simulink model "adc"  (R2019a)
settings: Solver=VariableStepAuto  StartTime=0.0  StopTime=500  RelTol=1e-3
libraries: xbsIndex_r4 x104, simulink x16
settings Model: Creator=qwerty40  LastModifiedBy=jackh
settings DataIOCC: ReturnWorkspaceOutputs=off
settings DebuggingCC: ArithmeticOperatorsInVariantConditions=warning
settings SFSimCC: SimUseLocalCustomCode=off
settings RTWCC: RTWUseLocalCustomCode=off
settings CodeAppCC: StateflowObjectComments=on

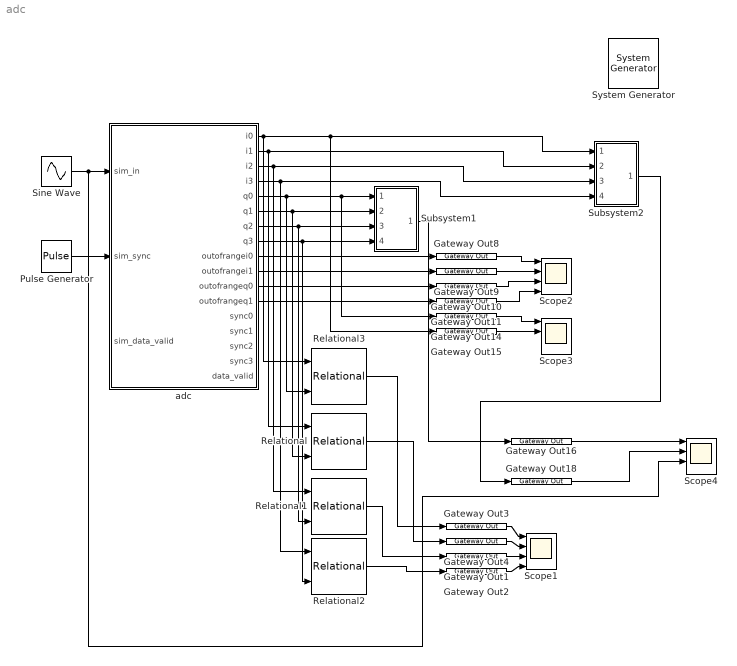
== system adc ==
  " System Generator" : xbsIndex_r4/ System Generator  Tag=genX  xilinxfamily=kintex7  part=xc7k325t  speed=-3  package=fbg676  synthesis_tool=Vivado  clock_wrapper=Clock Enables  directory=./netlist  proj_type=Vivado  Synth_file=Vivado Synthesis Defaults  Impl_file=Vivado Implementation Defaults  testbench=off  simulink_period=1  sysclk_period=10  dcm_input_clock_period=10  incr_netlist=off  trim_vbits=Everywhere in SubSystem  dbl_ovrd=According to Block Masks  core_generation=According to Block Masks  run_coregen=off  deprecated_control=off  eval_field=0  block_type=sysgen
  Gateway Out{1..4,8..11,14..16,18} (12 alike) : xbsIndex_r4/Gateway Out  inherit_from_input=off  hdl_port=on  rows=1  columns=1  UseAsDAC=off  DACChannel='1'  interface=None  automatic_assignment=on  address_offset=hex2dec('00')  intf_name=''  intf_description=''  timing_constraint=None  locs_specified=off  LOCs={}  io_standard={}  block_type=gatewayout
  Pulse Generator : DiscretePulseGenerator  Period=100
  Relational{,1..3} (4 alike) : xbsIndex_r4/Relational  mode=a=b  op_type=Bool  en=off  latency=1  dbl_ovrd=off  block_type=relational
  Scope{1..4} (4 alike) : Scope  NumInputPorts=4
  Sine Wave : Sin  SineType=Sample based  Amplitude=0.5  Frequency=pi / 30  Samples=100  SampleTime=1
  Subsystem1 : Subsystem
  Subsystem2 : Subsystem
  adc : Subsystem  Tag=xps:adc  mask(adc){adc_brd=adc0, adc_clk_rate=800, adc_interleave=off, sample_period=4}
      mask prompts: adc_brd "ADC board"; adc_clk_rate "ADC clock rate (MHz)"; adc_interleave "ADC interleave mode"; sample_period "Sample period"
      mask help: The ADC block converts analog inputs to digital outputs. Every clock cycle, the inputs are sampled and digitized to 8 bit binary point numbers in the range of [-1, 1) and are then output by the adc.
      mask init:
      | adc_mask;
      mask Help: eval('xlWeb([getenv(''MLIB_ROOT''), ''\doc\html\sys_adc\sys_adc.html''])')
      mask TypeOptions adc_brd: adc0 | adc1
  wires:
  Pulse Generator/1 -> adc/2(sim_sync)
  Gateway Out8/1 -> Scope2/1
  Gateway Out9/1 -> Scope2/2
  Gateway Out10/1 -> Scope2/3
  Gateway Out11/1 -> Scope2/4
  ? -> Scope3/4
  ? -> Scope3/3
  Gateway Out15/1 -> Scope3/2
  Gateway Out14/1 -> Scope3/1
  Gateway Out16/1 -> Scope4/1
  adc/1(i0) -> Relational3/1, Gateway Out15/1, Subsystem2/1(In1)
  adc/2(i1) -> Relational/1, Subsystem2/2(In2)
  adc/3(i2) -> Relational1/1, Subsystem2/3(In3)
  adc/4(i3) -> Relational2/1, Subsystem2/4(In4)
  Gateway Out18/1 -> Scope4/2
  adc/9(outofrangei0) -> Gateway Out8/1
  adc/10(outofrangei1) -> Gateway Out9/1
  adc/11(outofrangeq0) -> Gateway Out10/1
  adc/12(outofrangeq1) -> Gateway Out11/1
  Subsystem1/1(Out1) -> Gateway Out16/1
  Subsystem2/1(Out1) -> Gateway Out18/1
  adc/6(q1) -> Relational/2, Subsystem1/2(In2)
  adc/7(q2) -> Relational1/2, Subsystem1/3(In3)
  adc/8(q3) -> Relational2/2, Subsystem1/4(In4)
  adc/5(q0) -> Relational3/2, Subsystem1/1(In1), Gateway Out14/1
  Relational3/1 -> Gateway Out3/1
  Gateway Out3/1 -> Scope1/1
  Gateway Out4/1 -> Scope1/2
  Gateway Out1/1 -> Scope1/3
  Gateway Out2/1 -> Scope1/4
  Relational/1 -> Gateway Out4/1
  Relational1/1 -> Gateway Out1/1
  Relational2/1 -> Gateway Out2/1
  Sine Wave/1 -> Scope4/3, adc/1(sim_in)

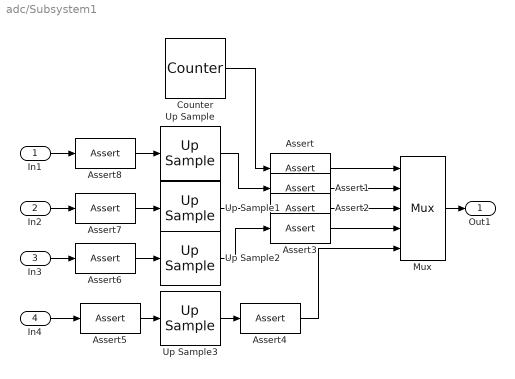
== system adc/Subsystem1 ==
  In1 : Inport
  In2 : Inport  Port=2
  In3 : Inport  Port=3
  In4 : Inport  Port=4
  Assert{,1..4} (5 alike) : xbsIndex_r4/Assert  assert_type=off  type_source=Explicitly  gui_display_data_type=Fixed-point  arith_type="Signed  (2's comp)"  n_bits=16  bin_pt=14  preci_type=Single  exp_width=8  frac_width=24  assert_rate=on  rate_source=Explicitly  period=1  output_port=on  block_type=assert
  Assert{5..8} (4 alike) : xbsIndex_r4/Assert  assert_type=off  type_source=Explicitly  gui_display_data_type=Fixed-point  arith_type="Signed  (2's comp)"  n_bits=16  bin_pt=14  preci_type=Single  exp_width=8  frac_width=24  assert_rate=on  rate_source=Explicitly  period=4  output_port=on  block_type=assert
  Counter : xbsIndex_r4/Counter  cnt_type=Free Running  cnt_to=Inf  operation=Up  start_count=0  cnt_by_val=1  arith_type=Unsigned  n_bits=2  bin_pt=0  load_pin=off  rst=off  en=off  explicit_period=on  period=1  use_behavioral_HDL=off  implementation=Fabric  dbl_ovrd=off  block_type=counter
  Mux : xbsIndex_r4/Mux  inputs=4  en=off  latency=1  precision=Full  arith_type=Unsigned  n_bits=16  bin_pt=14  quantization=Truncate  overflow=Wrap  dbl_ovrd=off  block_type=mux
  Up Sample{,1..3} (4 alike) : xbsIndex_r4/Up Sample  sample_ratio=4  copy_samples=on  en=off  latency=1  dbl_ovrd=off  block_type=usamp
  Out1 : Outport
  wires:
  Assert8/1 -> Up Sample/1
  Assert7/1 -> Up Sample1/1
  Assert6/1 -> Up Sample2/1
  Assert5/1 -> Up Sample3/1
  Counter/1 -> Assert/1
  Up Sample1/1 -> Assert2/1
  Mux/1 -> Out1/1
  In4/1 -> Assert5/1
  In2/1 -> Assert7/1
  In3/1 -> Assert6/1
  In1/1 -> Assert8/1
  Up Sample/1 -> Assert1/1
  Up Sample2/1 -> Assert3/1
  Up Sample3/1 -> Assert4/1
  Assert/1 -> Mux/1
  Assert1/1 -> Mux/2
  Assert2/1 -> Mux/3
  Assert3/1 -> Mux/4
  Assert4/1 -> Mux/5

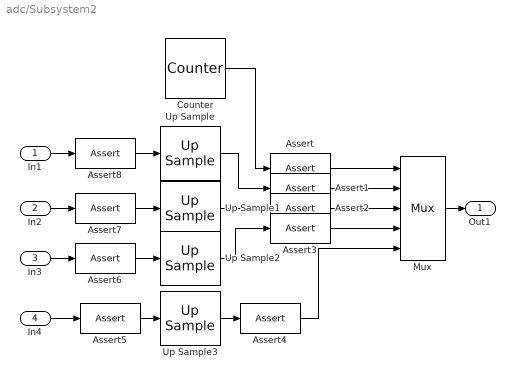
== system adc/Subsystem2 ==
  In1 : Inport
  In2 : Inport  Port=2
  In3 : Inport  Port=3
  In4 : Inport  Port=4
  Assert{,1..4} (5 alike) : xbsIndex_r4/Assert  assert_type=off  type_source=Explicitly  gui_display_data_type=Fixed-point  arith_type="Signed  (2's comp)"  n_bits=16  bin_pt=14  preci_type=Single  exp_width=8  frac_width=24  assert_rate=on  rate_source=Explicitly  period=1  output_port=on  block_type=assert
  Assert{5..8} (4 alike) : xbsIndex_r4/Assert  assert_type=off  type_source=Explicitly  gui_display_data_type=Fixed-point  arith_type="Signed  (2's comp)"  n_bits=16  bin_pt=14  preci_type=Single  exp_width=8  frac_width=24  assert_rate=on  rate_source=Explicitly  period=4  output_port=on  block_type=assert
  Counter : xbsIndex_r4/Counter  cnt_type=Free Running  cnt_to=Inf  operation=Up  start_count=0  cnt_by_val=1  arith_type=Unsigned  n_bits=2  bin_pt=0  load_pin=off  rst=off  en=off  explicit_period=on  period=1  use_behavioral_HDL=off  implementation=Fabric  dbl_ovrd=off  block_type=counter
  Mux : xbsIndex_r4/Mux  inputs=4  en=off  latency=1  precision=Full  arith_type=Unsigned  n_bits=16  bin_pt=14  quantization=Truncate  overflow=Wrap  dbl_ovrd=off  block_type=mux
  Up Sample{,1..3} (4 alike) : xbsIndex_r4/Up Sample  sample_ratio=4  copy_samples=on  en=off  latency=1  dbl_ovrd=off  block_type=usamp
  Out1 : Outport
  wires:
  Assert4/1 -> Mux/5
  Assert3/1 -> Mux/4
  Assert2/1 -> Mux/3
  Assert1/1 -> Mux/2
  Assert/1 -> Mux/1
  Up Sample3/1 -> Assert4/1
  Up Sample2/1 -> Assert3/1
  Up Sample/1 -> Assert1/1
  In1/1 -> Assert8/1
  In3/1 -> Assert6/1
  In2/1 -> Assert7/1
  In4/1 -> Assert5/1
  Mux/1 -> Out1/1
  Up Sample1/1 -> Assert2/1
  Counter/1 -> Assert/1
  Assert5/1 -> Up Sample3/1
  Assert6/1 -> Up Sample2/1
  Assert7/1 -> Up Sample1/1
  Assert8/1 -> Up Sample/1

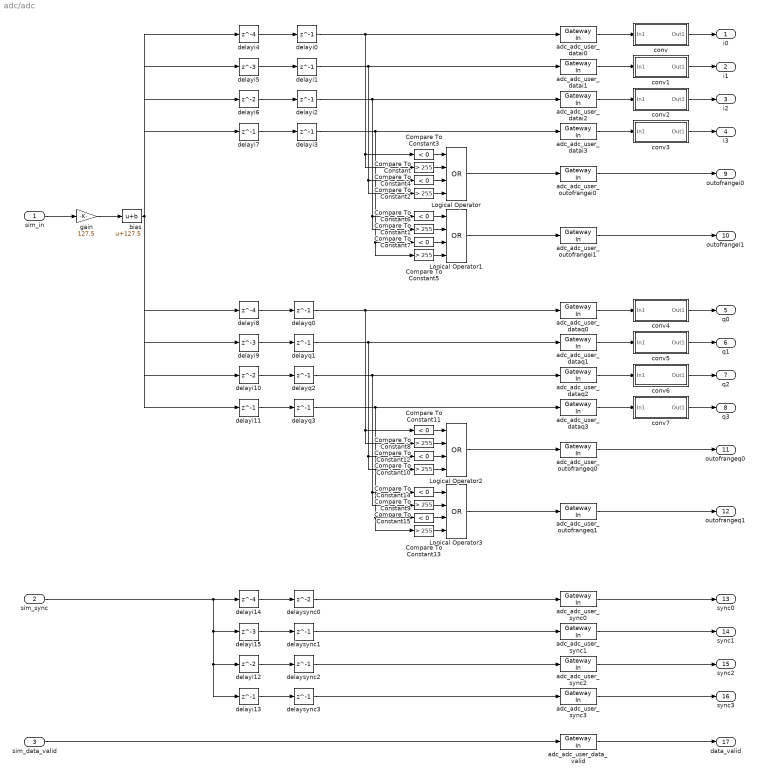
== system adc/adc ==
  sim_in : Inport  SampleTime=sample_period/4
  sim_sync : Inport  Port=2  SampleTime=sample_period/4
  sim_data_valid : Inport  Port=3  SampleTime=sample_period/4
  Compare To Constant{,1..2,5,8..10,13} (8 alike) : simulink/Logic and Bit Operations/Compare To Constant  relop=>  const=255  OutDataTypeStr=boolean  ZeroCross=off
  Compare To Constant{3..4,6..7,11..12,14..15} (8 alike) : simulink/Logic and Bit Operations/Compare To Constant  relop=<  const=0  OutDataTypeStr=boolean  ZeroCross=off
  Logical Operator{,1..3} (4 alike) : Logic  Operator=OR  Inputs=4  AllPortsSameDT=off  OutDataTypeStr=boolean
  adc_adc_user_data_valid : xbsIndex_r4/Gateway In  gui_display_data_type=Fixed-point  arith_type=Boolean  n_bits=8  bin_pt=0  preci_type=Single  exp_width=8  frac_width=24  rows=1  columns=1  quantization="Round  (unbiased: +/- Inf)"  overflow=Saturate  period=sample_period  UseAsADC=off  ADCChannel='1'  interface=None  automatic_assignment=on  address_offset=hex2dec('00')  intf_name=''  intf_description=''  default_value=0  timing_constraint=None  locs_specified=off  LOCs={}  io_standard={}  inherit_from_input=off  hdl_port=on  dbl_ovrd=off  block_type=gatewayin
      settings: infoedit="Gateway in block.  Converts inputs of type Simulink integer, double and fixed point to  Xilinx fixed point type.<P><P>Hardware notes:  In hardware these blocks become top level input ports."  xl_area=[0 0 0 0 8 0 0]  block_version=8.2.02
  adc_adc_user_datai{0..3} (4 alike) : xbsIndex_r4/Gateway In  gui_display_data_type=Fixed-point  arith_type=Unsigned  n_bits=8  bin_pt=0  preci_type=Single  exp_width=8  frac_width=24  rows=1  columns=1  quantization="Round  (unbiased: +/- Inf)"  overflow=Saturate  period=sample_period  UseAsADC=off  ADCChannel='1'  interface=None  automatic_assignment=on  address_offset=hex2dec('00')  intf_name=''  intf_description=''  default_value=0  timing_constraint=None  locs_specified=off  LOCs={}  io_standard={}  inherit_from_input=off  hdl_port=on  dbl_ovrd=off  block_type=gatewayin
      settings: infoedit="Gateway in block.  Converts inputs of type Simulink integer, double and fixed point to  Xilinx fixed point type.<P><P>Hardware notes:  In hardware these blocks become top level input ports."  xl_area=[0 0 0 0 8 0 0]  block_version=8.2.02
  adc_adc_user_dataq{0..3} (4 alike) : xbsIndex_r4/Gateway In  gui_display_data_type=Fixed-point  arith_type=Unsigned  n_bits=8  bin_pt=0  preci_type=Single  exp_width=8  frac_width=24  rows=1  columns=1  quantization="Round  (unbiased: +/- Inf)"  overflow=Saturate  period=sample_period  UseAsADC=off  ADCChannel='1'  interface=None  automatic_assignment=on  address_offset=hex2dec('00')  intf_name=''  intf_description=''  default_value=0  timing_constraint=None  locs_specified=off  LOCs={}  io_standard={}  inherit_from_input=off  hdl_port=on  dbl_ovrd=off  block_type=gatewayin
      settings: infoedit="Gateway in block.  Converts inputs of type Simulink integer, double and fixed point to  Xilinx fixed point type.<P><P>Hardware notes:  In hardware these blocks become top level input ports."  xl_area=[0 0 0 0 8 0 0]  block_version=8.2.02
  adc_adc_user_outofrangei0 : xbsIndex_r4/Gateway In  gui_display_data_type=Fixed-point  arith_type=Boolean  n_bits=8  bin_pt=0  preci_type=Single  exp_width=8  frac_width=24  rows=1  columns=1  quantization="Round  (unbiased: +/- Inf)"  overflow=Saturate  period=sample_period  UseAsADC=off  ADCChannel='1'  interface=None  automatic_assignment=on  address_offset=hex2dec('00')  intf_name=''  intf_description=''  default_value=0  timing_constraint=None  locs_specified=off  LOCs={}  io_standard={}  inherit_from_input=off  hdl_port=on  dbl_ovrd=off  block_type=gatewayin
      settings: infoedit="Gateway in block.  Converts inputs of type Simulink integer, double and fixed point to  Xilinx fixed point type.<P><P>Hardware notes:  In hardware these blocks become top level input ports."  xl_area=[0 0 0 0 8 0 0]  block_version=8.2.02
  adc_adc_user_outofrangei1 : xbsIndex_r4/Gateway In  gui_display_data_type=Fixed-point  arith_type=Boolean  n_bits=8  bin_pt=0  preci_type=Single  exp_width=8  frac_width=24  rows=1  columns=1  quantization="Round  (unbiased: +/- Inf)"  overflow=Saturate  period=sample_period  UseAsADC=off  ADCChannel='1'  interface=None  automatic_assignment=on  address_offset=hex2dec('00')  intf_name=''  intf_description=''  default_value=0  timing_constraint=None  locs_specified=off  LOCs={}  io_standard={}  inherit_from_input=off  hdl_port=on  dbl_ovrd=off  block_type=gatewayin
      settings: infoedit="Gateway in block.  Converts inputs of type Simulink integer, double and fixed point to  Xilinx fixed point type.<P><P>Hardware notes:  In hardware these blocks become top level input ports."  xl_area=[0 0 0 0 8 0 0]  block_version=8.2.02
  adc_adc_user_outofrangeq0 : xbsIndex_r4/Gateway In  gui_display_data_type=Fixed-point  arith_type=Boolean  n_bits=8  bin_pt=0  preci_type=Single  exp_width=8  frac_width=24  rows=1  columns=1  quantization="Round  (unbiased: +/- Inf)"  overflow=Saturate  period=sample_period  UseAsADC=off  ADCChannel='1'  interface=None  automatic_assignment=on  address_offset=hex2dec('00')  intf_name=''  intf_description=''  default_value=0  timing_constraint=None  locs_specified=off  LOCs={}  io_standard={}  inherit_from_input=off  hdl_port=on  dbl_ovrd=off  block_type=gatewayin
      settings: infoedit="Gateway in block.  Converts inputs of type Simulink integer, double and fixed point to  Xilinx fixed point type.<P><P>Hardware notes:  In hardware these blocks become top level input ports."  xl_area=[0 0 0 0 8 0 0]  block_version=8.2.02
  adc_adc_user_outofrangeq1 : xbsIndex_r4/Gateway In  gui_display_data_type=Fixed-point  arith_type=Boolean  n_bits=8  bin_pt=0  preci_type=Single  exp_width=8  frac_width=24  rows=1  columns=1  quantization="Round  (unbiased: +/- Inf)"  overflow=Saturate  period=sample_period  UseAsADC=off  ADCChannel='1'  interface=None  automatic_assignment=on  address_offset=hex2dec('00')  intf_name=''  intf_description=''  default_value=0  timing_constraint=None  locs_specified=off  LOCs={}  io_standard={}  inherit_from_input=off  hdl_port=on  dbl_ovrd=off  block_type=gatewayin
      settings: infoedit="Gateway in block.  Converts inputs of type Simulink integer, double and fixed point to  Xilinx fixed point type.<P><P>Hardware notes:  In hardware these blocks become top level input ports."  xl_area=[0 0 0 0 8 0 0]  block_version=8.2.02
  adc_adc_user_sync{0..3} (4 alike) : xbsIndex_r4/Gateway In  gui_display_data_type=Fixed-point  arith_type=Boolean  n_bits=8  bin_pt=0  preci_type=Single  exp_width=8  frac_width=24  rows=1  columns=1  quantization="Round  (unbiased: +/- Inf)"  overflow=Saturate  period=sample_period  UseAsADC=off  ADCChannel='1'  interface=None  automatic_assignment=on  address_offset=hex2dec('00')  intf_name=''  intf_description=''  default_value=0  timing_constraint=None  locs_specified=off  LOCs={}  io_standard={}  inherit_from_input=off  hdl_port=on  dbl_ovrd=off  block_type=gatewayin
      settings: infoedit="Gateway in block.  Converts inputs of type Simulink integer, double and fixed point to  Xilinx fixed point type.<P><P>Hardware notes:  In hardware these blocks become top level input ports."  xl_area=[0 0 0 0 8 0 0]  block_version=8.2.02
  bias : Bias  Bias=127.5  SaturateOnIntegerOverflow=on
  conv : Subsystem
  conv1 : Subsystem
  conv2 : Subsystem
  conv3 : Subsystem
  conv4 : Subsystem
  conv5 : Subsystem
  conv6 : Subsystem
  conv7 : Subsystem
  delayi{0..3,7,11,13} (7 alike) : Delay  DelayLength=1
  delayi10 : Delay
  delayi12 : Delay
  delayi14 : Delay  DelayLength=4
  delayi15 : Delay  DelayLength=3
  delayi4 : Delay  DelayLength=4
  delayi5 : Delay  DelayLength=3
  delayi6 : Delay
  delayi8 : Delay  DelayLength=4
  delayi9 : Delay  DelayLength=3
  delayq{0..3} (4 alike) : Delay  DelayLength=1
  delaysync0 : Delay
  delaysync1 : Delay  DelayLength=1
  delaysync2 : Delay  DelayLength=1
  delaysync3 : Delay  DelayLength=1
  gain : Gain  Gain=127.5  SaturateOnIntegerOverflow=on  OutDataTypeStr=Inherit: Same as input  ParamDataTypeStr=Inherit: Same as input
  i0 : Outport
  i1 : Outport  Port=2
  i2 : Outport  Port=3
  i3 : Outport  Port=4
  q0 : Outport  Port=5
  q1 : Outport  Port=6
  q2 : Outport  Port=7
  q3 : Outport  Port=8
  outofrangei0 : Outport  Port=9
  outofrangei1 : Outport  Port=10
  outofrangeq0 : Outport  Port=11
  outofrangeq1 : Outport  Port=12
  sync0 : Outport  Port=13
  sync1 : Outport  Port=14
  sync2 : Outport  Port=15
  sync3 : Outport  Port=16
  data_valid : Outport  Port=17
  wires:
  bias/1 -> delayi10/1, delayi9/1, delayi11/1, delayi8/1, delayi7/1, delayi6/1, delayi5/1, delayi4/1
  gain/1 -> bias/1
  sim_in/1 -> gain/1
  adc_adc_user_datai0/1 -> conv/1(In1)
  sim_data_valid/1 -> adc_adc_user_data_valid/1
  adc_adc_user_data_valid/1 -> data_valid/1
  adc_adc_user_sync3/1 -> sync3/1
  adc_adc_user_sync2/1 -> sync2/1
  delaysync3/1 -> adc_adc_user_sync3/1
  delaysync2/1 -> adc_adc_user_sync2/1
  delayi13/1 -> delaysync3/1
  delayi12/1 -> delaysync2/1
  adc_adc_user_sync1/1 -> sync1/1
  delaysync0/1 -> adc_adc_user_sync0/1
  delayi15/1 -> delaysync1/1
  delayi14/1 -> delaysync0/1
  sim_sync/1 -> delayi14/1, delayi15/1, delayi13/1, delayi12/1
  Logical Operator3/1 -> adc_adc_user_outofrangeq1/1
  Compare To Constant13/1 -> Logical Operator3/4
  Compare To Constant15/1 -> Logical Operator3/3
  Compare To Constant9/1 -> Logical Operator3/2
  Compare To Constant14/1 -> Logical Operator3/1
  Logical Operator2/1 -> adc_adc_user_outofrangeq0/1
  Compare To Constant10/1 -> Logical Operator2/4
  Compare To Constant12/1 -> Logical Operator2/3
  Compare To Constant8/1 -> Logical Operator2/2
  Compare To Constant11/1 -> Logical Operator2/1
  adc_adc_user_outofrangeq1/1 -> outofrangeq1/1
  adc_adc_user_outofrangeq0/1 -> outofrangeq0/1
  Logical Operator1/1 -> adc_adc_user_outofrangei1/1
  Compare To Constant5/1 -> Logical Operator1/4
  Compare To Constant7/1 -> Logical Operator1/3
  Compare To Constant1/1 -> Logical Operator1/2
  Compare To Constant6/1 -> Logical Operator1/1
  Logical Operator/1 -> adc_adc_user_outofrangei0/1
  Compare To Constant2/1 -> Logical Operator/4
  Compare To Constant4/1 -> Logical Operator/3
  Compare To Constant/1 -> Logical Operator/2
  Compare To Constant3/1 -> Logical Operator/1
  adc_adc_user_outofrangei1/1 -> outofrangei1/1
  delayq0/1 -> Compare To Constant8/1, Compare To Constant11/1, adc_adc_user_dataq0/1
  delayi8/1 -> delayq0/1
  delayi0/1 -> Compare To Constant3/1, Compare To Constant/1, adc_adc_user_datai0/1
  delayi5/1 -> delayi1/1
  delayi6/1 -> delayi2/1
  delayi7/1 -> delayi3/1
  delayi9/1 -> delayq1/1
  delayi10/1 -> delayq2/1
  delayi11/1 -> delayq3/1
  adc_adc_user_datai1/1 -> conv1/1(In1)
  adc_adc_user_datai2/1 -> conv2/1(In1)
  adc_adc_user_datai3/1 -> conv3/1(In1)
  adc_adc_user_outofrangei0/1 -> outofrangei0/1
  adc_adc_user_sync0/1 -> sync0/1
  conv/1(Out1) -> i0/1
  conv1/1(Out1) -> i1/1
  conv2/1(Out1) -> i2/1
  conv3/1(Out1) -> i3/1
  adc_adc_user_dataq0/1 -> conv4/1(In1)
  conv4/1(Out1) -> q0/1
  adc_adc_user_dataq1/1 -> conv5/1(In1)
  conv5/1(Out1) -> q1/1
  adc_adc_user_dataq2/1 -> conv6/1(In1)
  conv6/1(Out1) -> q2/1
  adc_adc_user_dataq3/1 -> conv7/1(In1)
  conv7/1(Out1) -> q3/1
  delayi4/1 -> delayi0/1
  delayi1/1 -> Compare To Constant4/1, Compare To Constant2/1, adc_adc_user_datai1/1
  delayi2/1 -> Compare To Constant1/1, Compare To Constant6/1, adc_adc_user_datai2/1
  delayi3/1 -> Compare To Constant5/1, Compare To Constant7/1, adc_adc_user_datai3/1
  delayq1/1 -> Compare To Constant10/1, Compare To Constant12/1, adc_adc_user_dataq1/1
  delayq2/1 -> Compare To Constant9/1, Compare To Constant14/1, adc_adc_user_dataq2/1
  delayq3/1 -> Compare To Constant13/1, Compare To Constant15/1, adc_adc_user_dataq3/1
  delaysync1/1 -> adc_adc_user_sync1/1

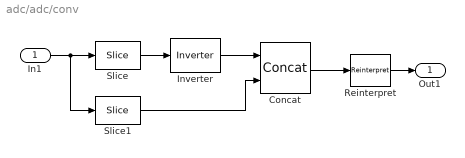
== system adc/adc/conv ==
  In1 : Inport
  Concat : xbsIndex_r4/Concat  num_inputs=2  dbl_ovrd=off  block_type=concat
      settings: block_version=8.2.02
  Inverter : xbsIndex_r4/Inverter  en=off  latency=0  dbl_ovrd=off  block_type=inv
      settings: xl_area=[0, 0, 0, 0, 0, 0, 0]  block_version=8.2.02
  Reinterpret : xbsIndex_r4/Reinterpret  force_arith_type=on  arith_type="Signed  (2's comp)"  force_bin_pt=on  bin_pt=7  block_type=reinterpret
      settings: infoedit="Changes signal type without altering the binary representation.   You can changed the signal between signed and unsigned, and relocate the binary point.<P><P>Hardware notes: In hardware this block costs nothing.<P><P>Example:  Suppose the input is 6 bits wide, signed, with 2 fractional bits, and the output is forced to unsigned with 0 fractional bits.  Then an input of -2.0 (1110.00 in binary 2's complement) becomes an output of 56 (111000 in binary)."  block_version=8.2.02
  Slice : xbsIndex_r4/Slice  nbits=1  boolean_output=off  mode=Upper Bit Location + Width  bit1=0  base1=MSB of Input  bit0=0  base0=LSB of Input  dbl_ovrd=off  block_type=slice
      settings: infoedit="Extracts a given range of bits from each input sample and presents it at the output.  The output type is ordinarily unsigned with binary point at zero, but can be Boolean when the slice is one bit wide.<P><P>Hardware notes: In hardware this block costs nothing."  block_version=8.2.02
  Slice1 : xbsIndex_r4/Slice  nbits=7  boolean_output=off  mode=Lower Bit Location + Width  bit1=0  base1=MSB of Input  bit0=0  base0=LSB of Input  dbl_ovrd=off  block_type=slice
      settings: infoedit="Extracts a given range of bits from each input sample and presents it at the output.  The output type is ordinarily unsigned with binary point at zero, but can be Boolean when the slice is one bit wide.<P><P>Hardware notes: In hardware this block costs nothing."  block_version=8.2.02
  Out1 : Outport
  wires:
  In1/1 -> Slice1/1, Slice/1
  Slice/1 -> Inverter/1
  Inverter/1 -> Concat/1
  Slice1/1 -> Concat/2
  Concat/1 -> Reinterpret/1
  Reinterpret/1 -> Out1/1

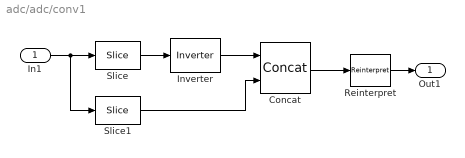
== system adc/adc/conv1 ==
  In1 : Inport
  Concat : xbsIndex_r4/Concat  num_inputs=2  dbl_ovrd=off  block_type=concat
      settings: block_version=8.2.02
  Inverter : xbsIndex_r4/Inverter  en=off  latency=0  dbl_ovrd=off  block_type=inv
      settings: xl_area=[0, 0, 0, 0, 0, 0, 0]  block_version=8.2.02
  Reinterpret : xbsIndex_r4/Reinterpret  force_arith_type=on  arith_type="Signed  (2's comp)"  force_bin_pt=on  bin_pt=7  block_type=reinterpret
      settings: infoedit="Changes signal type without altering the binary representation.   You can changed the signal between signed and unsigned, and relocate the binary point.<P><P>Hardware notes: In hardware this block costs nothing.<P><P>Example:  Suppose the input is 6 bits wide, signed, with 2 fractional bits, and the output is forced to unsigned with 0 fractional bits.  Then an input of -2.0 (1110.00 in binary 2's complement) becomes an output of 56 (111000 in binary)."  block_version=8.2.02
  Slice : xbsIndex_r4/Slice  nbits=1  boolean_output=off  mode=Upper Bit Location + Width  bit1=0  base1=MSB of Input  bit0=0  base0=LSB of Input  dbl_ovrd=off  block_type=slice
      settings: infoedit="Extracts a given range of bits from each input sample and presents it at the output.  The output type is ordinarily unsigned with binary point at zero, but can be Boolean when the slice is one bit wide.<P><P>Hardware notes: In hardware this block costs nothing."  block_version=8.2.02
  Slice1 : xbsIndex_r4/Slice  nbits=7  boolean_output=off  mode=Lower Bit Location + Width  bit1=0  base1=MSB of Input  bit0=0  base0=LSB of Input  dbl_ovrd=off  block_type=slice
      settings: infoedit="Extracts a given range of bits from each input sample and presents it at the output.  The output type is ordinarily unsigned with binary point at zero, but can be Boolean when the slice is one bit wide.<P><P>Hardware notes: In hardware this block costs nothing."  block_version=8.2.02
  Out1 : Outport
  wires:
  In1/1 -> Slice1/1, Slice/1
  Slice/1 -> Inverter/1
  Inverter/1 -> Concat/1
  Slice1/1 -> Concat/2
  Concat/1 -> Reinterpret/1
  Reinterpret/1 -> Out1/1

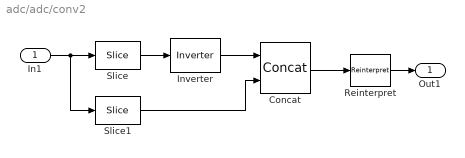
== system adc/adc/conv2 ==
  In1 : Inport
  Concat : xbsIndex_r4/Concat  num_inputs=2  dbl_ovrd=off  block_type=concat
      settings: block_version=8.2.02
  Inverter : xbsIndex_r4/Inverter  en=off  latency=0  dbl_ovrd=off  block_type=inv
      settings: xl_area=[0, 0, 0, 0, 0, 0, 0]  block_version=8.2.02
  Reinterpret : xbsIndex_r4/Reinterpret  force_arith_type=on  arith_type="Signed  (2's comp)"  force_bin_pt=on  bin_pt=7  block_type=reinterpret
      settings: infoedit="Changes signal type without altering the binary representation.   You can changed the signal between signed and unsigned, and relocate the binary point.<P><P>Hardware notes: In hardware this block costs nothing.<P><P>Example:  Suppose the input is 6 bits wide, signed, with 2 fractional bits, and the output is forced to unsigned with 0 fractional bits.  Then an input of -2.0 (1110.00 in binary 2's complement) becomes an output of 56 (111000 in binary)."  block_version=8.2.02
  Slice : xbsIndex_r4/Slice  nbits=1  boolean_output=off  mode=Upper Bit Location + Width  bit1=0  base1=MSB of Input  bit0=0  base0=LSB of Input  dbl_ovrd=off  block_type=slice
      settings: infoedit="Extracts a given range of bits from each input sample and presents it at the output.  The output type is ordinarily unsigned with binary point at zero, but can be Boolean when the slice is one bit wide.<P><P>Hardware notes: In hardware this block costs nothing."  block_version=8.2.02
  Slice1 : xbsIndex_r4/Slice  nbits=7  boolean_output=off  mode=Lower Bit Location + Width  bit1=0  base1=MSB of Input  bit0=0  base0=LSB of Input  dbl_ovrd=off  block_type=slice
      settings: infoedit="Extracts a given range of bits from each input sample and presents it at the output.  The output type is ordinarily unsigned with binary point at zero, but can be Boolean when the slice is one bit wide.<P><P>Hardware notes: In hardware this block costs nothing."  block_version=8.2.02
  Out1 : Outport
  wires:
  In1/1 -> Slice1/1, Slice/1
  Slice/1 -> Inverter/1
  Inverter/1 -> Concat/1
  Slice1/1 -> Concat/2
  Concat/1 -> Reinterpret/1
  Reinterpret/1 -> Out1/1

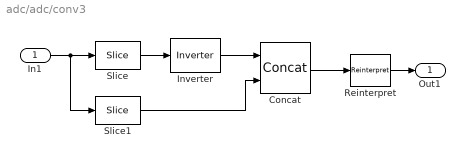
== system adc/adc/conv3 ==
  In1 : Inport
  Concat : xbsIndex_r4/Concat  num_inputs=2  dbl_ovrd=off  block_type=concat
      settings: block_version=8.2.02
  Inverter : xbsIndex_r4/Inverter  en=off  latency=0  dbl_ovrd=off  block_type=inv
      settings: xl_area=[0, 0, 0, 0, 0, 0, 0]  block_version=8.2.02
  Reinterpret : xbsIndex_r4/Reinterpret  force_arith_type=on  arith_type="Signed  (2's comp)"  force_bin_pt=on  bin_pt=7  block_type=reinterpret
      settings: infoedit="Changes signal type without altering the binary representation.   You can changed the signal between signed and unsigned, and relocate the binary point.<P><P>Hardware notes: In hardware this block costs nothing.<P><P>Example:  Suppose the input is 6 bits wide, signed, with 2 fractional bits, and the output is forced to unsigned with 0 fractional bits.  Then an input of -2.0 (1110.00 in binary 2's complement) becomes an output of 56 (111000 in binary)."  block_version=8.2.02
  Slice : xbsIndex_r4/Slice  nbits=1  boolean_output=off  mode=Upper Bit Location + Width  bit1=0  base1=MSB of Input  bit0=0  base0=LSB of Input  dbl_ovrd=off  block_type=slice
      settings: infoedit="Extracts a given range of bits from each input sample and presents it at the output.  The output type is ordinarily unsigned with binary point at zero, but can be Boolean when the slice is one bit wide.<P><P>Hardware notes: In hardware this block costs nothing."  block_version=8.2.02
  Slice1 : xbsIndex_r4/Slice  nbits=7  boolean_output=off  mode=Lower Bit Location + Width  bit1=0  base1=MSB of Input  bit0=0  base0=LSB of Input  dbl_ovrd=off  block_type=slice
      settings: infoedit="Extracts a given range of bits from each input sample and presents it at the output.  The output type is ordinarily unsigned with binary point at zero, but can be Boolean when the slice is one bit wide.<P><P>Hardware notes: In hardware this block costs nothing."  block_version=8.2.02
  Out1 : Outport
  wires:
  In1/1 -> Slice1/1, Slice/1
  Slice/1 -> Inverter/1
  Inverter/1 -> Concat/1
  Slice1/1 -> Concat/2
  Concat/1 -> Reinterpret/1
  Reinterpret/1 -> Out1/1

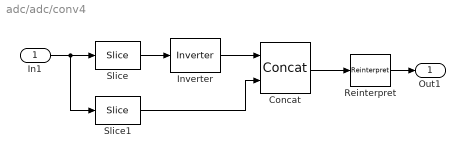
== system adc/adc/conv4 ==
  In1 : Inport
  Concat : xbsIndex_r4/Concat  num_inputs=2  dbl_ovrd=off  block_type=concat
      settings: block_version=8.2.02
  Inverter : xbsIndex_r4/Inverter  en=off  latency=0  dbl_ovrd=off  block_type=inv
      settings: xl_area=[0, 0, 0, 0, 0, 0, 0]  block_version=8.2.02
  Reinterpret : xbsIndex_r4/Reinterpret  force_arith_type=on  arith_type="Signed  (2's comp)"  force_bin_pt=on  bin_pt=7  block_type=reinterpret
      settings: infoedit="Changes signal type without altering the binary representation.   You can changed the signal between signed and unsigned, and relocate the binary point.<P><P>Hardware notes: In hardware this block costs nothing.<P><P>Example:  Suppose the input is 6 bits wide, signed, with 2 fractional bits, and the output is forced to unsigned with 0 fractional bits.  Then an input of -2.0 (1110.00 in binary 2's complement) becomes an output of 56 (111000 in binary)."  block_version=8.2.02
  Slice : xbsIndex_r4/Slice  nbits=1  boolean_output=off  mode=Upper Bit Location + Width  bit1=0  base1=MSB of Input  bit0=0  base0=LSB of Input  dbl_ovrd=off  block_type=slice
      settings: infoedit="Extracts a given range of bits from each input sample and presents it at the output.  The output type is ordinarily unsigned with binary point at zero, but can be Boolean when the slice is one bit wide.<P><P>Hardware notes: In hardware this block costs nothing."  block_version=8.2.02
  Slice1 : xbsIndex_r4/Slice  nbits=7  boolean_output=off  mode=Lower Bit Location + Width  bit1=0  base1=MSB of Input  bit0=0  base0=LSB of Input  dbl_ovrd=off  block_type=slice
      settings: infoedit="Extracts a given range of bits from each input sample and presents it at the output.  The output type is ordinarily unsigned with binary point at zero, but can be Boolean when the slice is one bit wide.<P><P>Hardware notes: In hardware this block costs nothing."  block_version=8.2.02
  Out1 : Outport
  wires:
  In1/1 -> Slice1/1, Slice/1
  Slice/1 -> Inverter/1
  Inverter/1 -> Concat/1
  Slice1/1 -> Concat/2
  Concat/1 -> Reinterpret/1
  Reinterpret/1 -> Out1/1

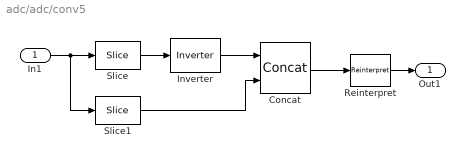
== system adc/adc/conv5 ==
  In1 : Inport
  Concat : xbsIndex_r4/Concat  num_inputs=2  dbl_ovrd=off  block_type=concat
      settings: block_version=8.2.02
  Inverter : xbsIndex_r4/Inverter  en=off  latency=0  dbl_ovrd=off  block_type=inv
      settings: xl_area=[0, 0, 0, 0, 0, 0, 0]  block_version=8.2.02
  Reinterpret : xbsIndex_r4/Reinterpret  force_arith_type=on  arith_type="Signed  (2's comp)"  force_bin_pt=on  bin_pt=7  block_type=reinterpret
      settings: infoedit="Changes signal type without altering the binary representation.   You can changed the signal between signed and unsigned, and relocate the binary point.<P><P>Hardware notes: In hardware this block costs nothing.<P><P>Example:  Suppose the input is 6 bits wide, signed, with 2 fractional bits, and the output is forced to unsigned with 0 fractional bits.  Then an input of -2.0 (1110.00 in binary 2's complement) becomes an output of 56 (111000 in binary)."  block_version=8.2.02
  Slice : xbsIndex_r4/Slice  nbits=1  boolean_output=off  mode=Upper Bit Location + Width  bit1=0  base1=MSB of Input  bit0=0  base0=LSB of Input  dbl_ovrd=off  block_type=slice
      settings: infoedit="Extracts a given range of bits from each input sample and presents it at the output.  The output type is ordinarily unsigned with binary point at zero, but can be Boolean when the slice is one bit wide.<P><P>Hardware notes: In hardware this block costs nothing."  block_version=8.2.02
  Slice1 : xbsIndex_r4/Slice  nbits=7  boolean_output=off  mode=Lower Bit Location + Width  bit1=0  base1=MSB of Input  bit0=0  base0=LSB of Input  dbl_ovrd=off  block_type=slice
      settings: infoedit="Extracts a given range of bits from each input sample and presents it at the output.  The output type is ordinarily unsigned with binary point at zero, but can be Boolean when the slice is one bit wide.<P><P>Hardware notes: In hardware this block costs nothing."  block_version=8.2.02
  Out1 : Outport
  wires:
  In1/1 -> Slice1/1, Slice/1
  Slice/1 -> Inverter/1
  Inverter/1 -> Concat/1
  Slice1/1 -> Concat/2
  Concat/1 -> Reinterpret/1
  Reinterpret/1 -> Out1/1

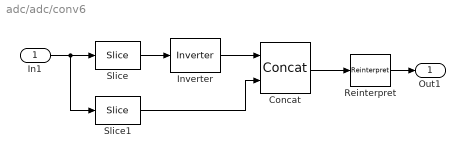
== system adc/adc/conv6 ==
  In1 : Inport
  Concat : xbsIndex_r4/Concat  num_inputs=2  dbl_ovrd=off  block_type=concat
      settings: block_version=8.2.02
  Inverter : xbsIndex_r4/Inverter  en=off  latency=0  dbl_ovrd=off  block_type=inv
      settings: xl_area=[0, 0, 0, 0, 0, 0, 0]  block_version=8.2.02
  Reinterpret : xbsIndex_r4/Reinterpret  force_arith_type=on  arith_type="Signed  (2's comp)"  force_bin_pt=on  bin_pt=7  block_type=reinterpret
      settings: infoedit="Changes signal type without altering the binary representation.   You can changed the signal between signed and unsigned, and relocate the binary point.<P><P>Hardware notes: In hardware this block costs nothing.<P><P>Example:  Suppose the input is 6 bits wide, signed, with 2 fractional bits, and the output is forced to unsigned with 0 fractional bits.  Then an input of -2.0 (1110.00 in binary 2's complement) becomes an output of 56 (111000 in binary)."  block_version=8.2.02
  Slice : xbsIndex_r4/Slice  nbits=1  boolean_output=off  mode=Upper Bit Location + Width  bit1=0  base1=MSB of Input  bit0=0  base0=LSB of Input  dbl_ovrd=off  block_type=slice
      settings: infoedit="Extracts a given range of bits from each input sample and presents it at the output.  The output type is ordinarily unsigned with binary point at zero, but can be Boolean when the slice is one bit wide.<P><P>Hardware notes: In hardware this block costs nothing."  block_version=8.2.02
  Slice1 : xbsIndex_r4/Slice  nbits=7  boolean_output=off  mode=Lower Bit Location + Width  bit1=0  base1=MSB of Input  bit0=0  base0=LSB of Input  dbl_ovrd=off  block_type=slice
      settings: infoedit="Extracts a given range of bits from each input sample and presents it at the output.  The output type is ordinarily unsigned with binary point at zero, but can be Boolean when the slice is one bit wide.<P><P>Hardware notes: In hardware this block costs nothing."  block_version=8.2.02
  Out1 : Outport
  wires:
  In1/1 -> Slice1/1, Slice/1
  Slice/1 -> Inverter/1
  Inverter/1 -> Concat/1
  Slice1/1 -> Concat/2
  Concat/1 -> Reinterpret/1
  Reinterpret/1 -> Out1/1

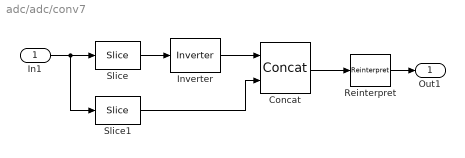
== system adc/adc/conv7 ==
  In1 : Inport
  Concat : xbsIndex_r4/Concat  num_inputs=2  dbl_ovrd=off  block_type=concat
      settings: block_version=8.2.02
  Inverter : xbsIndex_r4/Inverter  en=off  latency=0  dbl_ovrd=off  block_type=inv
      settings: xl_area=[0, 0, 0, 0, 0, 0, 0]  block_version=8.2.02
  Reinterpret : xbsIndex_r4/Reinterpret  force_arith_type=on  arith_type="Signed  (2's comp)"  force_bin_pt=on  bin_pt=7  block_type=reinterpret
      settings: infoedit="Changes signal type without altering the binary representation.   You can changed the signal between signed and unsigned, and relocate the binary point.<P><P>Hardware notes: In hardware this block costs nothing.<P><P>Example:  Suppose the input is 6 bits wide, signed, with 2 fractional bits, and the output is forced to unsigned with 0 fractional bits.  Then an input of -2.0 (1110.00 in binary 2's complement) becomes an output of 56 (111000 in binary)."  block_version=8.2.02
  Slice : xbsIndex_r4/Slice  nbits=1  boolean_output=off  mode=Upper Bit Location + Width  bit1=0  base1=MSB of Input  bit0=0  base0=LSB of Input  dbl_ovrd=off  block_type=slice
      settings: infoedit="Extracts a given range of bits from each input sample and presents it at the output.  The output type is ordinarily unsigned with binary point at zero, but can be Boolean when the slice is one bit wide.<P><P>Hardware notes: In hardware this block costs nothing."  block_version=8.2.02
  Slice1 : xbsIndex_r4/Slice  nbits=7  boolean_output=off  mode=Lower Bit Location + Width  bit1=0  base1=MSB of Input  bit0=0  base0=LSB of Input  dbl_ovrd=off  block_type=slice
      settings: infoedit="Extracts a given range of bits from each input sample and presents it at the output.  The output type is ordinarily unsigned with binary point at zero, but can be Boolean when the slice is one bit wide.<P><P>Hardware notes: In hardware this block costs nothing."  block_version=8.2.02
  Out1 : Outport
  wires:
  In1/1 -> Slice1/1, Slice/1
  Slice/1 -> Inverter/1
  Inverter/1 -> Concat/1
  Slice1/1 -> Concat/2
  Concat/1 -> Reinterpret/1
  Reinterpret/1 -> Out1/1
